simulink model "Simple_OFDM_Model_Start"  (R2026a)
settings: Solver=ode3  StopTime=2  FixedStep=0.5  EnableMultiTasking=on
PreLoadFcn:
  | nSubCar=12;
  | nOFDMSym=1;
libraries: dspxfrm3 x2, matrix_library x1, commrandsrc3 x1, commdigbbndam3 x1
settings Model: Creator=thua3267  LastModifiedBy=vuong
settings HardwareCC: ProdHWDeviceType=32-bit Generic

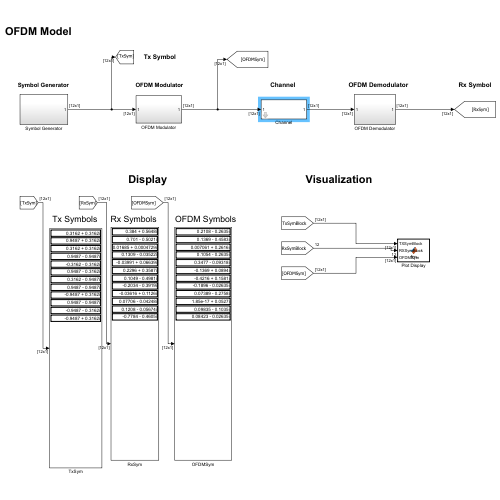
[thumbnail: Simulink's stored preview of the top-level diagram]
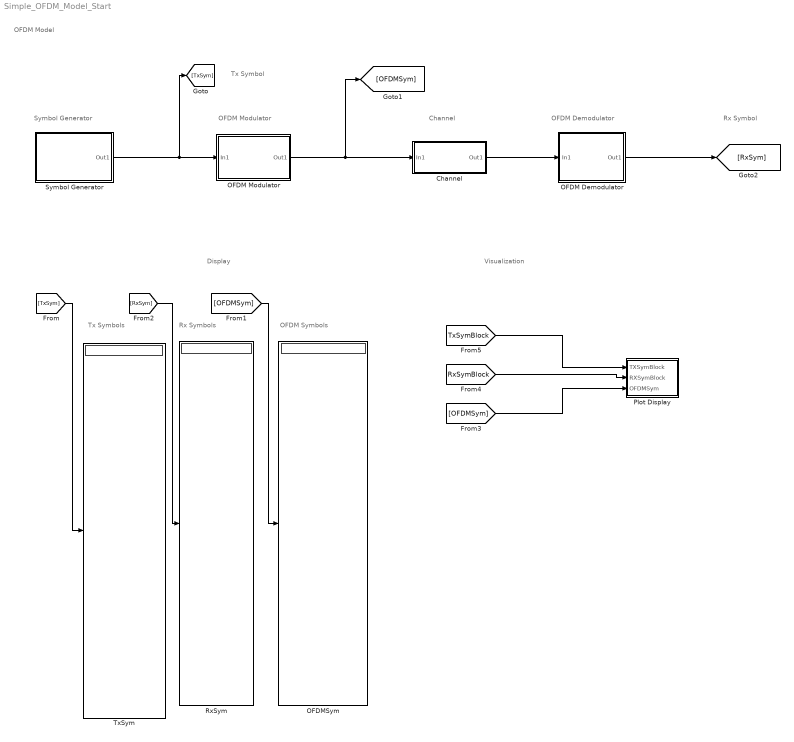
== system Simple_OFDM_Model_Start ==
  note: Visualization
  note: Symbol Generator
  note: OFDM Model
  note: OFDM Symbols
  note: Rx Symbols
  note: Tx Symbols
  note: Display
  note: OFDM Modulator
  note: Channel
  note: OFDM Demodulator
  note: Rx Symbol
  note: Tx Symbol
  Channel : Subsystem  Tag=Ideal upconverter, Channel and downconverter  mask{ChanSelect=2}
      mask prompts: ChanSelect "Channel Selection"
      mask help:
      | Channel Selection Parameter
      | 1 ideal channel
      | 2 frequency selective channel A
      | 3 frequency selective channel B
      | 4 frequency selective channel LTEA
      | 5 frequency selective channel LTEB
  OFDM Demodulator : Subsystem
  OFDM Modulator : Subsystem
  OFDMSym : Display
  Plot Display : MATLAB Function  TreatAsAtomicUnit=on
  RxSym : Display
  Symbol Generator : Subsystem
  TxSym : Display
  wires:
  [TxSym] -> TxSym/1
  [OFDMSym] -> OFDMSym/1
  [RxSym] -> RxSym/1
  [TxSymBlock] -> Plot Display/1(TXSymBlock)
  [RxSymBlock] -> Plot Display/2(RXSymBlock)
  OFDM Modulator/1(Out1) -> [OFDMSym], Channel/1(In1)
  Channel/1(Out1) -> OFDM Demodulator/1(In1)
  OFDM Demodulator/1(Out1) -> [RxSym]
  [OFDMSym] -> Plot Display/3(OFDMSym)
  Symbol Generator/1(Out1) -> [TxSym], OFDM Modulator/1(In1)

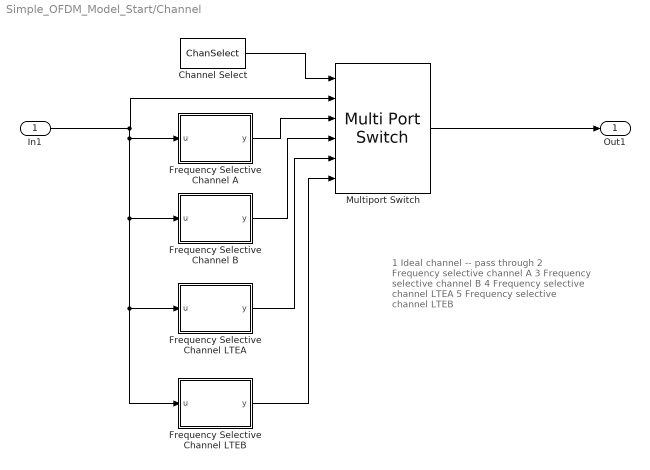
== system Simple_OFDM_Model_Start/Channel ==
  note: 1 Ideal channel  --  pass through
      | 2 Frequency selective channel A
      | 3 Frequency selective channel B
      | 4 Frequency selective channel LTEA
      | 5 Frequency selective channel LTEB
  In1 : Inport
  Channel Select : Constant  Value=ChanSelect  VectorParams1D=off  OutMin=1  OutMax=5  OutDataTypeStr=Inherit: Inherit via back propagation
  Frequency Selective Channel A : MATLAB Function  TreatAsAtomicUnit=on
  Frequency Selective Channel B : MATLAB Function  TreatAsAtomicUnit=on
  Frequency Selective Channel LTEA : MATLAB Function  TreatAsAtomicUnit=on
  Frequency Selective Channel LTEB : MATLAB Function  TreatAsAtomicUnit=on
  Multiport Switch : MultiPortSwitch  Inputs=5  SaturateOnIntegerOverflow=off  InputSameDT=off
  Out1 : Outport  VectorParamsAs1DForOutWhenUnconnected=off
  wires:
  In1/1 -> Frequency Selective Channel B/1(u), Frequency Selective Channel LTEB/1(u), Frequency Selective Channel LTEA/1(u), Frequency Selective Channel A/1(u), Multiport Switch/2
  Multiport Switch/1 -> Out1/1
  Channel Select/1 -> Multiport Switch/1
  Frequency Selective Channel A/1(y) -> Multiport Switch/3
  Frequency Selective Channel LTEB/1(y) -> Multiport Switch/6
  Frequency Selective Channel LTEA/1(y) -> Multiport Switch/5
  Frequency Selective Channel B/1(y) -> Multiport Switch/4

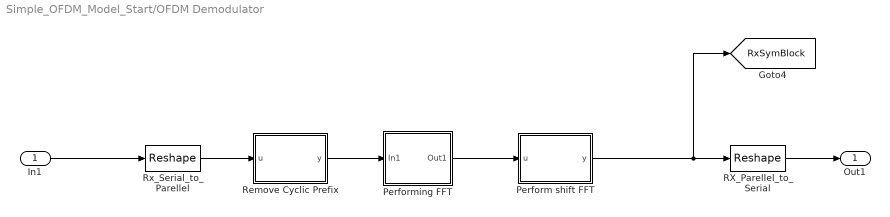
== system Simple_OFDM_Model_Start/OFDM Demodulator ==
  In1 : Inport
  " RX_Parellel_to_Serial" : Reshape  OutputDimensionality=Column vector (2-D)
  Perform shift FFT : MATLAB Function  TreatAsAtomicUnit=on
  Performing FFT : Subsystem
  Remove Cyclic Prefix : MATLAB Function  TreatAsAtomicUnit=on
  Rx_Serial_to_Parellel : Reshape  OutputDimensionality=Customize  OutputDimensions=[nSubCar nOFDMSym]
  Out1 : Outport  VectorParamsAs1DForOutWhenUnconnected=off
  tag scope: RxSymBlock=global
  wires:
  " RX_Parellel_to_Serial"/1 -> Out1/1
  In1/1 -> Rx_Serial_to_Parellel/1
  Rx_Serial_to_Parellel/1 -> Remove Cyclic Prefix/1(u)
  Performing FFT/1(Out1) -> Perform shift FFT/1(u)
  Remove Cyclic Prefix/1(y) -> Performing FFT/1(In1)
  Perform shift FFT/1(y) -> " RX_Parellel_to_Serial"/1, [RxSymBlock]

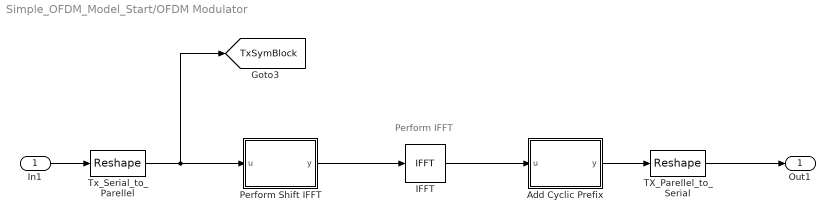
== system Simple_OFDM_Model_Start/OFDM Modulator ==
  note: Perform IFFT
  In1 : Inport
  " TX_Parellel_to_Serial" : Reshape  OutputDimensionality=Column vector (2-D)
  Add Cyclic Prefix : MATLAB Function  TreatAsAtomicUnit=on
  IFFT : dspxfrm3/IFFT  FFTImplementation=Auto  CompMethod=Table lookup  TableOpt=NEW  TableOptActive=Speed  BitRevOrder=off  cs_in=off  Normalize=on  InheritFFTLength=on  FFTLength=128  WrapInput=on  mode=Complex  outSamplingMode=Sample based  roundingMode=Floor  overflowMode=off  firstCoeffDataTypeStr=Inherit: Same word length as input  firstCoeffLastDataTypeStr=Inherit: Same word length as input  outputMin=[]  outputMax=[]
  Perform Shift IFFT : MATLAB Function  TreatAsAtomicUnit=on
  Tx_Serial_to_Parellel : Reshape  OutputDimensionality=Customize  OutputDimensions=[nSubCar nOFDMSym]
  Out1 : Outport  VectorParamsAs1DForOutWhenUnconnected=off
  tag scope: TxSymBlock=global
  wires:
  Tx_Serial_to_Parellel/1 -> Perform Shift IFFT/1(u), [TxSymBlock]
  " TX_Parellel_to_Serial"/1 -> Out1/1
  Add Cyclic Prefix/1(y) -> " TX_Parellel_to_Serial"/1
  In1/1 -> Tx_Serial_to_Parellel/1
  IFFT/1 -> Add Cyclic Prefix/1(u)
  Perform Shift IFFT/1(y) -> IFFT/1

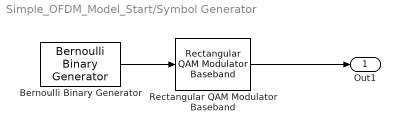
== system Simple_OFDM_Model_Start/Symbol Generator ==
  Bernoulli Binary Generator : commrandsrc3/Bernoulli Binary Generator  ProbabilityOfZero=0.5  SeedSource=Auto  Seed=0  SampleTime=1  SamplesPerFrame=nOFDMSym*nSubCar*4  OutputDataType=single  SimulateUsing=Interpreted execution
  Rectangular QAM Modulator Baseband : commdigbbndam3/Rectangular QAM Modulator Baseband  M=16  InType=Bit  Enc=Gray  Mapping=[0:15]  PowType=Average Power  MinDist=2  AvgPow=1  PeakPow=1  Ph=0  outDtype=double  outWordLen=16  outUDDataType=sfix(16)  outFracLenMode=Best precision  outFracLen=15  outDataTypeStr=double  outLastDataTypeStr=double
  Out1 : Outport  VectorParamsAs1DForOutWhenUnconnected=off
  wires:
  Bernoulli Binary Generator/1 -> Rectangular QAM Modulator Baseband/1
  Rectangular QAM Modulator Baseband/1 -> Out1/1

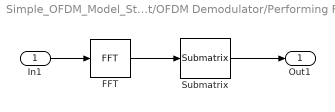
== system Simple_OFDM_Model_Start/OFDM Demodulator/Performing FFT ==
  In1 : Inport
  FFT : dspxfrm3/FFT  FFTImplementation=Auto  CompMethod=Table lookup  TableOpt=NEW  TableOptActive=Speed  BitRevOrder=off  Normalize=off  InheritFFTLength=on  FFTLength=64  WrapInput=on  roundingMode=Floor  overflowMode=off  firstCoeffDataTypeStr=Inherit: Same word length as input  firstCoeffLastDataTypeStr=Inherit: Same word length as input  outputMin=[]  outputMax=[]
  Submatrix : matrix_library/Submatrix  RowSpan=Range of rows  RowStartMode=First  RowStartIndex=1  RowEndMode=Index  RowEndIndex=nSubCar  ColSpan=Range of columns  ColStartMode=First  ColStartIndex=1  ColEndMode=Last  ColEndIndex=1
  Out1 : Outport  VectorParamsAs1DForOutWhenUnconnected=off
  wires:
  FFT/1 -> Submatrix/1
  In1/1 -> FFT/1
  Submatrix/1 -> Out1/1

== matlab function Simple_OFDM_Model_Start/Plot Display ==
  data: TXSymBlock input; RXSymBlock input; OFDMSym input; nOFDMSym parameter
function fcn(TXSymBlock, RXSymBlock, OFDMSym, nOFDMSym)
%% parameters
enabled = 1;           % enable plot
maxQAMSymbol = 2;      % symbol amplitude
nSubCar=12;            % maximum carriers to be plotted

%nOFDMSym;        % from workspace:  the number of symbols sent

%%
 coder.extrinsic('subplot','stem', 'plot','sprintf','movegui','iptwindowalign');
 
 if enabled
    figure(1);
    %movegui(figure(1),'northwest')
    for subIdx = 1:nSubCar,
        subplot(3,4,subIdx);
        plot(real(TXSymBlock(subIdx,:)),imag(TXSymBlock(subIdx,:)),'x');
        axis([-maxQAMSymbol maxQAMSymbol -maxQAMSymbol maxQAMSymbol]); axis square
        title(sprintf('TX SubCar %d',subIdx));
        grid on
    end %for subIdx

    figure(3);
    %iptwindowalign(figure(2),'right',figure(3),'left');
    stem((0:length(OFDMSym)-1),abs(OFDMSym));
    xlabel('time')
    title(sprintf('Time-Domain Symbols (for %d OFDM symbols)',nOFDMSym));
    
    
    figure(2);
    %movegui(figure(2),'north')
    %iptwindowalign(figure(1),'right',figure(2),'left');
    for subIdx = 1:nSubCar,
        subplot(3,4,subIdx); 
        plot(real(RXSymBlock(subIdx,:)),imag(RXSymBlock(subIdx,:)),'ro');
        axis([-maxQAMSymbol maxQAMSymbol -maxQAMSymbol maxQAMSymbol]); axis square
        title(sprintf('RX SubCar %d',subIdx));
        grid on
    end %for subIdx
    

end

== matlab function Simple_OFDM_Model_Start/Channel/Frequency Selective Channel A ==
  data: u input; y output
function y = freqSelChanA(u)
%#codegen
% Create frequency selective channel
b = firpm(4,[0 .2 .4 1],[1 0.01 0.01 1]);
y=filter(b,1,u);

== matlab function Simple_OFDM_Model_Start/OFDM Modulator/Add Cyclic Prefix ==
  data: u input; y output
function y = addCycPrefix(u)
%your code here
y=u;

== matlab function Simple_OFDM_Model_Start/OFDM Demodulator/Remove Cyclic Prefix ==
  data: u input; y output
function y = rmCycPref(u)
%your code here
y=u;

== matlab function Simple_OFDM_Model_Start/Channel/Frequency Selective Channel LTEA ==
  data: u input; y output
function y = freqSelChanLTEA(u)
%#codegen
% Create frequency selective channel
% LTE Downlink Physical Layer Parameters
% Channel Bandwidth 5 MHz, FFT size 512, Sample frequency 7.68

% Create frequency selective channel
b = firpm(24,[0 .2 .4 1],[1 0.02 0.02 1]);
y=filter(b,1,u);

== matlab function Simple_OFDM_Model_Start/Channel/Frequency Selective Channel LTEB ==
  data: u input; y output
function y = freqSelChanLTEB(u)
%#codegen
% Create frequency selective channel
% LTE Downlink Physical Layer Parameters
% Channel Bandwidth 10MHz, FFT size 1024, Sample frequency 15.36MHz
b = firpm(60,[0 .25 .35 1],[1 0.02 0.02 1]);
y=filter(b,1,u);

== matlab function Simple_OFDM_Model_Start/Channel/Frequency Selective Channel B ==
  data: u input; y output
function y = freqSelChanB(u)
%#codegen
% Create frequency selective channel
b = firpm(6,[0 .2 .4 1],[1 0.01 0.01 1]);
y=filter(b,1,u);

== matlab function Simple_OFDM_Model_Start/OFDM Modulator/Perform Shift IFFT ==
  data: u input; y output
function y = shiftIFFT(u)
y=ifftshift(u);

== matlab function Simple_OFDM_Model_Start/OFDM Demodulator/Perform shift FFT ==
  data: u input; y output
function y = shiftFFT(u)
y=fftshift(u);
